simulink model "scheme_L2"  (R2025b)
settings: Solver=ode4  StartTime=0.0  StopTime=12  FixedStep=0.001  RelTol=1e-3
settings Model: Creator=kiselyov.semen  LastModifiedBy=kiselyov.semen

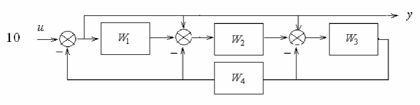
[thumbnail: Simulink's stored preview of the top-level diagram]
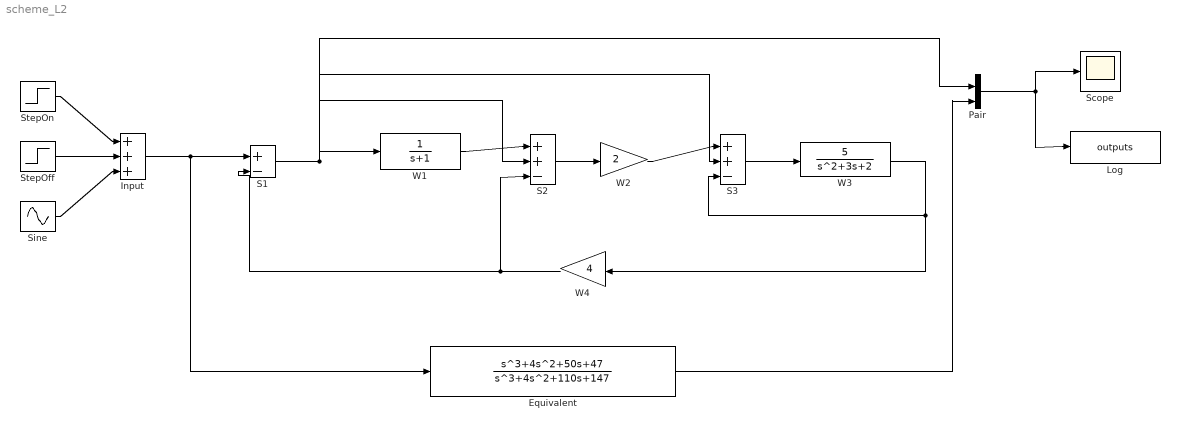
== system scheme_L2 ==
  StepOn : Step  Time=1  Before=0  After=1  SampleTime=0
  StepOff : Step  Time=1.05  Before=0  After=0  SampleTime=0
  Sine : Sin  Amplitude=0  Frequency=1  SampleTime=0
  Input : Sum  Inputs=+++
  S1 : Sum  Inputs=+-
  W1 : TransferFcn  Numerator=[1]  Denominator=[1 1]
  S2 : Sum  Inputs=++-
  W2 : Gain  Gain=2
  S3 : Sum  Inputs=++-
  W3 : TransferFcn  Numerator=[5]  Denominator=[1 3 2]
  W4 : Gain  Gain=4
  Equivalent : TransferFcn  Numerator=[1 4 50 47]  Denominator=[1 4 110 147]
  Pair : Mux  Inputs=2
  Scope : Scope
  Log : ToWorkspace  VariableName=outputs  SaveFormat=Timeseries  SampleTime=-1
  wires:
  StepOn/1 -> Input/1
  StepOff/1 -> Input/2
  Sine/1 -> Input/3
  Input/1 -> S1/1, Equivalent/1
  S1/1 -> W1/1, S2/2, S3/2, Pair/1
  W1/1 -> S2/1
  S2/1 -> W2/1
  W2/1 -> S3/1
  S3/1 -> W3/1
  W3/1 -> W4/1, S3/3
  W4/1 -> S1/2, S2/3
  Equivalent/1 -> Pair/2
  Pair/1 -> Scope/1, Log/1
